simulink model "SHRKIM002_Optimisation"  (R2026a)
settings: Solver=VariableStepAuto  StopTime=inf  MaxStep=0.04
InitFcn:
  | % Robot params
  | r_w = (67.60 / 2) / 1000; % wheel radius in m
  | d = (83 + 12.5 + 12.5) / 1000; % wheel centre-centre distance (width)
  | a = 33.275 / 1000; % IMU to wheel axle distance
  | 
  | % Motor params
  | k = 0.0192;
  | tau = 0.1718;
  | k_bodge = 3;
  | tau_bodge = 0.4;
  | 
  | noiseScalar = 1;
  | 
  | %control loop update rate
  | dt_loop = 0.02;
  | dt_sim = 0.005;
  | dt_plot = 0.1;
  | 
  | waypoint_matrix = centerlineTrack('SaoPaulo.csv');
model workspace (MAT data in the model file):
  d : Simulink.Parameter (value not decoded)
  dphi_limit : Simulink.Parameter (value not decoded)
  dt_sim : Simulink.Parameter (value not decoded)
  l_robot : Simulink.Parameter (value not decoded)
  m_robot : Simulink.Parameter (value not decoded)
  mpc1 : object (value not decoded)
  mpc_opt : object (value not decoded)
  nlobj : nlmpc (value not decoded)
  no_points : Simulink.Parameter (value not decoded)
  r_w : Simulink.Parameter (value not decoded)
  robot_half_w : Simulink.Parameter (value not decoded)
  sample_f : Simulink.Parameter (value not decoded)
  track_buffer : Simulink.Parameter (value not decoded)
  track_width : Simulink.Parameter (value not decoded)
  waypoint_gain : Simulink.Parameter (value not decoded)
values from neighbouring files (symbols this model uses):
  dphi_limit = 9.72    [controlNMPC.m]
symbols that are objects in the model workspace (value not decoded): l_robot, m_robot, no_points, robot_half_w, sample_f, track_buffer, track_width, waypoint_gain
undefined symbols (not defined in the file or in its folder): DiscIntNeverNeededParam
libraries: simulink x12, dspstat3 x6, slpidlib x2, mpclib x2, robotalgslib x1
(part 2 of 2)

== matlab function SHRKIM002_Optimisation/Robot Navigation & Control/Pose Estimator/MATLAB Function ==
  settings: updateMethod=DISCRETE  sampleTime=0.02
  data: v input; px_est output; psi_dot input; py_est output; psi_est output; dT input; pose_est_xy output; waypoints input
function [px_est, py_est, psi_est, pose_est_xy] = poseEstimator(v, psi_dot, dT, waypoints)

persistent T
if( isempty(T) )
    % at start find waypoints to set starting angle

    % use first and fifth waypoint
    w1 = waypoints(:,1);
    w2 = waypoints(:,5);

    % initial heading angle
    psi_init = atan2(w2(2) - w1(2), w2(1) - w1(1));

    % transformation matrix to start set to face the track
    T = [cos(psi_init), -sin(psi_init), w1(1);
        sin(psi_init), cos(psi_init), w1(2);
        0, 0, 1];
end


delta_psi = psi_dot * dT;

% checking if the angle is big enough so that there is no dividing by 0 error
if abs(psi_dot) > 1e-4

    R = [cos(delta_psi), -sin(delta_psi);
        sin(delta_psi),  cos(delta_psi)];

    J = [sin(delta_psi)/delta_psi,     (cos(delta_psi)-1)/delta_psi;
        (1-cos(delta_psi))/delta_psi, sin(delta_psi)/delta_psi];

    T_inc = [R, J*[v; 0]*dT; 0, 0 ,1];
    
else 
    T_inc = [cos(delta_psi), -sin(delta_psi), v * cos(delta_psi) * dT; 
             sin(delta_psi),  cos(delta_psi), v * sin(delta_psi) * dT;
             0 0 1];
end 

T = T*T_inc;

px_est  = T(1, 3);
py_est  = T(2, 3);
psi_est = atan2(T(2,1),T(1,1));
pose_est_xy = [px_est; py_est];

end

== matlab function SHRKIM002_Optimisation/2Wh. Robot/2Wh. Kinematics/MATLAB Function ==
  settings: updateMethod=DISCRETE
  data: waypoints input; dpx input; dpsi input; t output; psi output
function [t,psi] = updatePose(waypoints, dpx, dpsi)

persistent T;

if( isempty(T) )
    % at start find waypoints to set starting angle

    % use first and fifth waypoint
    w1 = waypoints(:,1);
    w2 = waypoints(:,5);

    % initial heading angle
    psi_init = atan2(w2(2) - w1(2), w2(1) - w1(1));

    % transformation matrix to start set to face the track
    T = [cos(psi_init), -sin(psi_init), w1(1);
        sin(psi_init), cos(psi_init), w1(2);
        0, 0, 1];
end

R = [cos(dpsi) -sin(dpsi);
      sin(dpsi)  cos(dpsi)];

if( abs(dpsi)<1e-5 )
    J = eye(2);
else
    J = [sin(dpsi)/(dpsi)     (cos(dpsi)-1)/(dpsi);
        (1-cos(dpsi))/(dpsi) sin(dpsi)/(dpsi)   ];
end

T_inc = [R J*[dpx 0]'; 0 0 1]; 
T = T*T_inc;

t = T(1:2,3);
psi = atan2(T(2,1),T(1,1));
end

== matlab function SHRKIM002_Optimisation/Robot Navigation & Control/Feedback Controller/Pure Pursuit/Switches/MATLAB Function ==
  data: pose_est_x input; e_lat output; pose_est_y input; p_des input; psi_des input; psi_est input; e_psi output
function [e_lat, e_psi] = calc_error(pose_est_x, pose_est_y, p_des, psi_des, psi_est)
    
% Global difference
    dx = pose_est_x - p_des(1);
    dy = pose_est_y - p_des(2);
    
    % Local (path bound) lateral difference
    e_lat = -sin(psi_des) * dx + cos(psi_des) * dy;
    
    % Properly wrapped heading error
    e_psi = atan2(sin(psi_est - psi_des), cos(psi_est - psi_des));
end

== matlab function SHRKIM002_Optimisation/Robot Navigation & Control/Feedback Controller/NMPC/Lateral Error Calculation ==
  data: pose_est_x input; pose_est_y input; e_lat output; p_des input; psi_des input; psi_est input; e_psi output
function [e_lat, e_psi] = calc_error(pose_est_x, pose_est_y, p_des, psi_des, psi_est)

    % Global difference
    dx = pose_est_x - p_des(1);
    dy = pose_est_y - p_des(2);
    
    % Local (path bound) lateral difference
    e_lat = -sin(psi_des) * dx + cos(psi_des) * dy;

    e_psi = atan2(sin(psi_est-psi_des),cos(psi_est - psi_des));
end

== matlab function SHRKIM002_Optimisation/Robot Navigation & Control/Trajectory Generator/Splines Trajectory Function ==
  data: Waypoints input; no_points parameter; p_des_array output; pose_est_xy input size=[2 1]; p_des output size=[2 1]; psi_des output size=1; kappa_des output size=1; index output; kappa_max output; dk_max output; n_jumps output; s_des output; v_lim_des output; dphi_limit parameter; sample_f parameter; r_w parameter; d parameter; T_pure_cent output; K_tot output; kappa_prev output
function [p_des_array, p_des, psi_des, kappa_des, index, kappa_max, dk_max, n_jumps, s_des, v_lim_des, T_pure_cent, K_tot, kappa_prev] = splines(Waypoints, no_points, pose_est_xy, dphi_limit, sample_f, r_w, d)
% Cubic Spline with arc length parameterisation

persistent p_array psi_array kappa_array kmax dkmax nj s_array vlim_array index_prev n_window T_pc Ktot ds_s kappa_sm
if isempty(p_array)
    [p_array, psi_array, kappa_array] = buildtrack(Waypoints, no_points);
    % find maximum curvature
    kmax = max(abs(kappa_array));
    dk = abs(diff(kappa_array)); 
    % find biggest jump between neighbouring samples
    dkmax = max(dk);
    nj = sum(dk > 0.5); % jumps larger than 0.5

    % true arc length,not waypoint sections
    s_array = [0, cumsum(sqrt(sum(diff(p_array,1,2).^2,1)))];

    ds_seg = diff(s_array);

    % total amount the robot turns over one lap
    Ktot = sum(abs(kappa_array(1:end-1)) .* ds_seg);
    % fastest lap if robot exactly on centerline
    T_pc = (s_array(end) + (d/2)*Ktot)/(r_w*dphi_limit);

    % path space between sampples
    ds_s = s_array(end)/(no_points-1);
    % smoothed curvature for racing-line reference only (moving average, wraps at lap end)
    w = 41; 
    h = (w-1)/2;
    kern = ones(1,w)/w;
    kp   = [kappa_array(end-h+1:end), kappa_array, kappa_array(1:h)];
    kappa_sm = conv(kp, kern, 'valid');          % same length as kappa_array

    % wheel-sat lim top speed on straight
    v_max_f = r_w*dphi_limit;
    % top speed at each point that keeps outer turning wheel in sat lim 
    v_max_out= v_max_f ./(1 + abs(kappa_array)*d/2);

    Ts = 1/sample_f;
    ds= s_array(end)/(no_points-1);
    % no. of path samples robot can do in one control step at top speed +1
    n_ticks = ceil(v_max_f*Ts/ds) + 1;
    vlim_array = v_max_out;
    for j = 1:no_points
        % last point within reach during step
        j_last = min(j+n_ticks, no_points);
        vmin = v_max_out(j);
        for k = j+1:j_last
            vmin = min(vmin, v_max_out(k));
        end
        % lowest final speed limit before controller updates (so robot slows
        % before taking a corner instead of slows inside the corner)
        vlim_array(j) = vmin;
    end

    index_prev = 1;
    % how many ticks robot should look on either side of point (plus safety margin) 
    n_window = 5*n_ticks + 10;

end

% upper and lower window so it stays in array
window_lower = max(1, index_prev - n_window);
window_upper = min(no_points, index_prev + n_window);

dmin = inf; 
index = index_prev;
% center of window on last ctrl step's point
% check in window and find closest point's index
for j = window_lower:window_upper
    squ_dist_j = (p_array(1,j)-pose_est_xy(1))^2 + (p_array(2,j)-pose_est_xy(2))^2;
    if squ_dist_j < dmin 
        dmin = squ_dist_j; 
        index = j; 
    end
end

index_prev = index;

p_des = p_array(:, index);
p_des_array = p_array;
psi_des = psi_array(index);
kappa_des = kappa_array(index);
s_des = s_array(index);
v_lim_des = vlim_array(index);
kappa_max = kmax;
dk_max  = dkmax;
n_jumps = nj;
T_pure_cent = T_pc;
K_tot  = Ktot;

% prediction horizon
P = 50;
step = v_lim_des/(sample_f*ds_s);
% future indices, wraps at lap end
idx = mod(round(index - 1 + (1:P)'*step), no_points) + 1; 
kappa_prev = reshape(kappa_sm(idx), P, 1);
end



% build track ahead of time to stop it from constantly rebuilding


function [p, psi, kappa] = buildtrack(Waypoints, no_points)


% Number of points to travel through
N = size(Waypoints, 2);

ds = zeros(1, N-1);
for i = 1:N-1
    ds(i) = norm(Waypoints(:,i+1) - Waypoints(:,i));
end

% running total of the elements
s_cum = [0, cumsum(ds)];
s_tot = s_cum(end);
% physical distance along track
s_steps = linspace(0, s_tot, no_points);

u_tangent = zeros(2, N);

for i = 1:N
    if i == 1
        tangent = Waypoints(:, 2) - Waypoints(:, 1);
    elseif i == N
        tangent = Waypoints(:, N) - Waypoints(:, N-1);
    else
        tangent = Waypoints(:, i+1) - Waypoints(:, i-1);
    end
    u_tangent(:,i) = tangent / norm(tangent);
end

p = zeros(2, no_points);  
dp = zeros(2, no_points);  
ddp = zeros(2, no_points);  
psi = zeros(1, no_points);  
kappa = zeros(1, no_points);

% Which segment each sample belongs to
seg = discretize(s_steps, s_cum);
% include the final point
seg(end) = N - 1;

for j = 1:no_points 

    s_index = seg(j);
    dS = ds(s_index);

    % % local normalised distance along segment
    s_l = s_steps(j) - s_cum(s_index);

    P0 = Waypoints(:, s_index);
    T0 = u_tangent(:, s_index);
    P1 = Waypoints(:, s_index+1);
    T1 = u_tangent(:, s_index+1);


    a0 = P0;
    a1 = T0;
    a2 = (3*(P1 - P0) - (2*T0 + T1)*dS) / dS.^2;
    a3 = (2*(P0 - P1) + (T0 + T1)*dS) / dS.^3;

    p(:, j) = a0 + a1*s_l + a2*s_l.^2 + a3*s_l.^3;
    dp(:, j) = a1 + 2*a2*s_l + 3*a3*s_l.^2;
    ddp(:, j) = 2*a2 + 6*a3*s_l;

    psi(j)   = atan2(dp(2,j), dp(1,j));
    kappa(j) = (dp(1,j)*ddp(2,j) - dp(2,j)*ddp(1,j)) / norm(dp(:,j))^3;
end
end
